simulink model "EXP3_Alamouti_21_Student"  (R2024a)
settings: Solver=FixedStepDiscrete  StartTime=0.0  StopTime=inf  RelTol=1e-3
PreLoadFcn:
  | EbNo = 5;
  | maxNumErrs = 100;
  | maxNumBits = 1e5;
undefined symbols (not defined in the file or in its folder): doppler
libraries: commchan3 x3, commdigbbndpm3 x2, commrandsrc3 x1, commsink2 x1
Description:
  | OSTBC over 3x2 Rayleigh fading channel
settings Model: Creator=The MathWorks Inc.  LastModifiedBy=yliu5829
settings SolverCC: AlgebraicLoopSolver=TrustRegion
settings DataIOCC: LimitDataPoints=on  SaveFormat=Array  SignalLoggingSaveFormat=ModelDataLogs  ReturnWorkspaceOutputs=off
settings OptimizationCC: DefaultParameterBehavior=Inlined  ExpressionDepthLimit=2147483647  LifeSpan=inf
settings DebuggingCC: UnderspecifiedInitializationDetection=Classic  MergeDetectMultiDrivingBlocksExec=none  SolverPrmCheckMsg=warning  FcnCallInpInsideContextMsg=warning  UnconnectedInputMsg=warning  UnconnectedOutputMsg=warning  UnconnectedLineMsg=warning  StateNameClashWarn=warning  SFUnexpectedBacktrackingDiag=warning  SFNoUnconditionalDefaultTransitionDiag=warning  SFExecutionAtInitializationDiag=none  ArithmeticOperatorsInVariantConditions=warning
settings HardwareCC: ProdBitPerPointer=32  ProdBitPerSizeT=32  ProdBitPerPtrDiffT=32  ProdLargestAtomicFloat=None  ProdIntDivRoundTo=Undefined  ProdEndianess=Unspecified  ProdWordSize=32  ProdHWDeviceType=32-bit Generic
settings ModelReferenceCC: EnableRefExpFcnMdlSchedulingChecks=on  PropagateSignalLabelsOutOfModel=off
settings SFSimCC: SimUseLocalCustomCode=off  CustomCodeUndefinedFunction=UseInterfaceOnly
settings RTWCC: RTWUseLocalCustomCode=off  GPUComputeCapability=3.5
settings CodeAppCC: StateflowObjectComments=on
settings GRTTargetCC: TargetLangStandard=C89/C90 (ANSI)  CombineOutputUpdateFcns=off  GRTInterface=on
settings ConfigComp: CovMetricSettings=dw  CovSaveCumulativeToWorkspaceVar=on  CovSaveSingleToWorkspaceVar=on  CovExternalEMLEnable=off  CovSFcnEnable=off

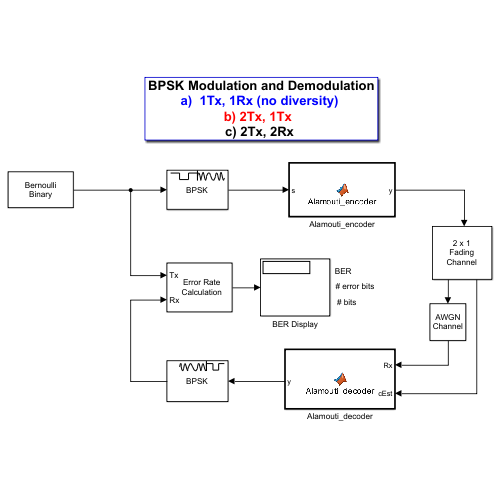
[thumbnail: Simulink's stored preview of the top-level diagram]
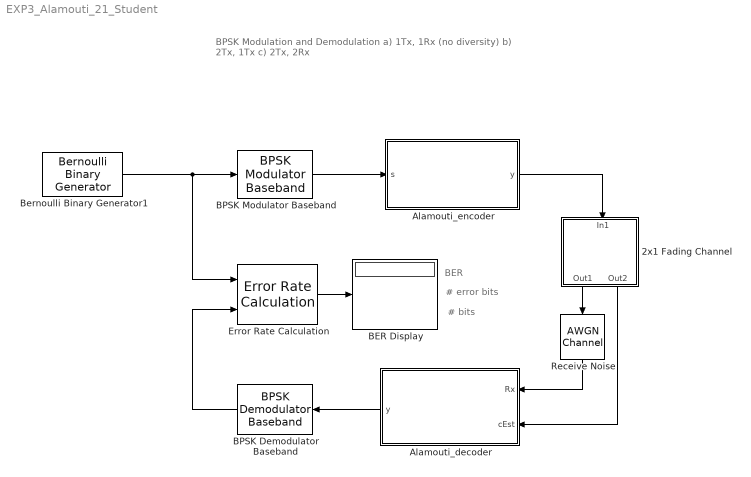
== system EXP3_Alamouti_21_Student ==
  note: BER
  note: # error bits
  note: # bits
  note: BPSK Modulation and Demodulation
      | a) 1Tx, 1Rx (no diversity)
      | b) 2Tx, 1Tx
      | c) 2Tx, 2Rx
  2x1 Fading Channel : Subsystem
      mask Display: disp('2 x 1\nFading\nChannel');
  Alamouti_decoder : MATLAB Function  TreatAsAtomicUnit=on
  Alamouti_encoder : MATLAB Function  TreatAsAtomicUnit=on
  BER Display : Display
  BPSK Demodulator Baseband : commdigbbndpm3/BPSK Demodulator Baseband  DecType=Hard decision  VarSource=Dialog  Variance=1  Ph=0  outDtype=boolean  derotateFactorWordLen=16  derotateFactorDataTypeStr=Inherit: Same word length as input  derotateFactorLastDataTypeStr=Inherit: Same word length as input
  BPSK Modulator Baseband : commdigbbndpm3/BPSK Modulator Baseband  Ph=0  outDtype=double  outWordLen=16  outUDDataType=sfix(16)  outFracLenMode=Best precision  outFracLen=15  outDataTypeStr=double  outLastDataTypeStr=double
  Bernoulli Binary Generator1 : commrandsrc3/Bernoulli Binary Generator  ProbabilityOfZero=.5  SeedSource=Parameter  Seed=61  SampleTime=1e-3  SamplesPerFrame=2  OutputDataType=boolean  SimulateUsing=Interpreted execution
  Error Rate Calculation : commsink2/Error Rate Calculation  N=0  st_delay=0  cp_mode=Entire frame  subframe=[]  PMode=Port  WsName=ErrorVec  RsMode2=off  stop=on  numErr=maxNumErrs  maxBits=maxNumBits
  Receive Noise : commchan3/AWGN Channel  LegacyMode=on  NoiseMethod="Signal to noise ratio  (SNR)"  noiseMode="Signal to noise ratio  (Eb/No)"  EbNo=EbNo  EsNo=5  SNR=EbNo - 10*log10(3)  BitsPerSymbol=1  SignalPower=2  SamplesPerSymbol=1  SymbolPeriod=1e-3  VarianceSource=Parameter  Variance=1  RandomStream=Global stream  Seed=188  SimulateUsing=Code generation
  wires:
  Bernoulli Binary Generator1/1 -> BPSK Modulator Baseband/1, Error Rate Calculation/1
  BPSK Modulator Baseband/1 -> Alamouti_encoder/1(s)
  Alamouti_encoder/1(y) -> 2x1 Fading Channel/1(In1)
  BPSK Demodulator Baseband/1 -> Error Rate Calculation/2
  Alamouti_decoder/1(y) -> BPSK Demodulator Baseband/1
  Error Rate Calculation/1 -> BER Display/1
  2x1 Fading Channel/1(Out1) -> Receive Noise/1
  2x1 Fading Channel/2(Out2) -> Alamouti_decoder/2(cEst)
  Receive Noise/1 -> Alamouti_decoder/1(Rx)

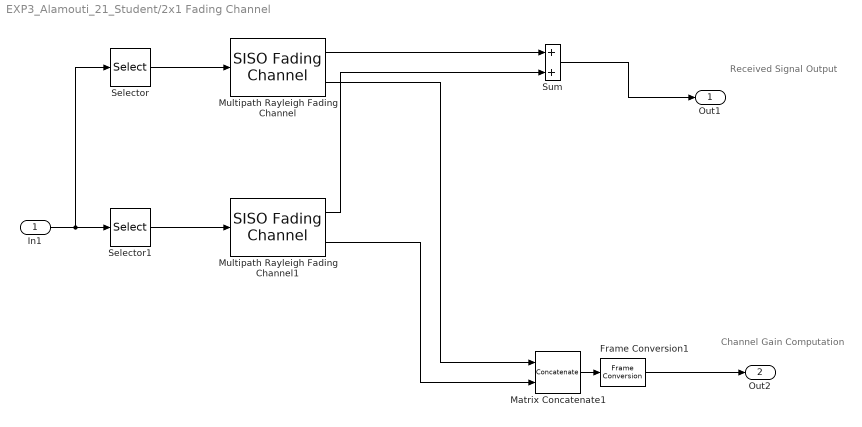
== system EXP3_Alamouti_21_Student/2x1 Fading Channel ==
  note: Received Signal Output
  note: Channel Gain Computation
  In1 : Inport
  Frame Conversion1 : FrameConversion  OutFrame=Sample-based
  Matrix Concatenate1 : Concatenate  Mode=Multidimensional array  ConcatenateDimension=2
  Multipath Rayleigh Fading Channel : commchan3/SISO Fading Channel  InheritSampleRate=on  SampleRate=1  PathDelays=0  AveragePathGains=0  NormalizePathGains=on  FadingDistribution=Rayleigh  KFactor=3  DirectPathDopplerShift=0  DirectPathInitialPhase=0  MaximumDopplerShift=3  DopplerSpectrum=doppler('Jakes')  RandomStream=mt19937ar with seed  Seed=12345  PathGainsOutputPort=on  ChannelFilterDelayOutputPort=off  SimulateUsing=Interpreted execution  Visualization=Off  PathsForDopplerDisplay=1  SamplesToDisplay=25%
  Multipath Rayleigh Fading Channel1 : commchan3/SISO Fading Channel  InheritSampleRate=on  SampleRate=1  PathDelays=0  AveragePathGains=0  NormalizePathGains=on  FadingDistribution=Rayleigh  KFactor=3  DirectPathDopplerShift=0  DirectPathInitialPhase=0  MaximumDopplerShift=3  DopplerSpectrum=doppler('Jakes')  RandomStream=mt19937ar with seed  Seed=24680  PathGainsOutputPort=on  ChannelFilterDelayOutputPort=off  SimulateUsing=Interpreted execution  Visualization=Off  PathsForDopplerDisplay=1  SamplesToDisplay=25%
  Selector : Selector  NumberOfDimensions=2  InputPortWidth=3  IndexOptions=Select all,Index vector (dialog)  Indices=-1,1  OutputSizes=1
  Selector1 : Selector  NumberOfDimensions=2  InputPortWidth=3  IndexOptions=Select all,Index vector (dialog)  Indices=-1,2  OutputSizes=1
  Sum : Sum
  Out1 : Outport  VectorParamsAs1DForOutWhenUnconnected=off
  Out2 : Outport  Port=2  VectorParamsAs1DForOutWhenUnconnected=off
  wires:
  In1/1 -> Selector1/1, Selector/1
  Multipath Rayleigh Fading Channel1/1 -> Sum/2
  Multipath Rayleigh Fading Channel/1 -> Sum/1
  Multipath Rayleigh Fading Channel1/2 -> Matrix Concatenate1/2
  Multipath Rayleigh Fading Channel/2 -> Matrix Concatenate1/1
  Selector1/1 -> Multipath Rayleigh Fading Channel1/1
  Selector/1 -> Multipath Rayleigh Fading Channel/1
  Sum/1 -> Out1/1
  Matrix Concatenate1/1 -> Frame Conversion1/1
  Frame Conversion1/1 -> Out2/1

== matlab function EXP3_Alamouti_21_Student/Alamouti_encoder ==
  data: s input; y output
function y = Alamouti_encoder(s)
%OSTBC Encoding Algorithms
y = [s,s];

== matlab function EXP3_Alamouti_21_Student/Alamouti_decoder ==
  data: Rx input; y output; cEst input
function y = Alamouti_decoder(Rx, cEst)
%Alamouti  decoding
y = Rx ;
mag = sum(sum((abs(cEst.^2))));
y = y./mag;
